simulink model "structure_track_side"  (R2026b)
settings: Solver=VariableStepAuto
model mask{side=1 left}
  mask prompts: side "Track side"
undefined symbols (not defined in the file or in its folder): P
libraries: fl_lib x11, nesl_utility x6
settings Model: Creator=aomar  LastModifiedBy=aomar

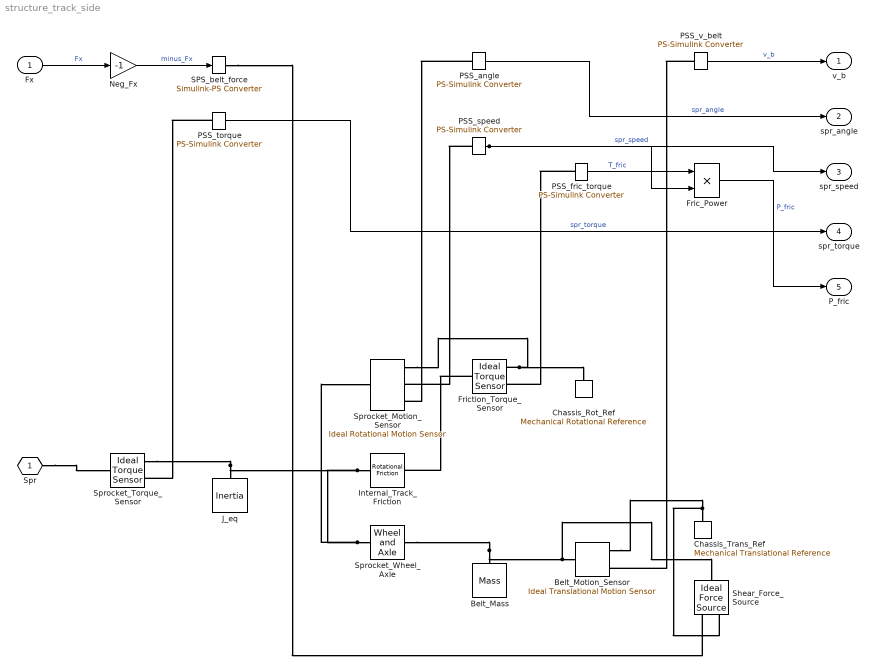
== system structure_track_side ==
  Fx : Inport
  Belt_Mass : fl_lib/Mechanical/Translational Elements/Mass  mass=P.structure.track.m_belt kg  num_ports=foundation.enum.numPorts2.one  v_specify=off  v_priority=High  v=0 m/s  v_nominal_specify=off  v_nominal_value=1  v_nominal_unit=m/s  f_specify=off  f_priority=None  f=0 N  f_nominal_specify=off  f_nominal_value=1  f_nominal_unit=N
  Belt_Motion_Sensor : fl_lib/Mechanical/Mechanical Sensors/Ideal Translational Motion Sensor  reference=foundation.enum.MeasurementReference.difference  acceleration_port=false  velocity_port=true  position_port=false  offset=0 m
  Chassis_Rot_Ref : fl_lib/Mechanical/Rotational Elements/Mechanical Rotational Reference
  Chassis_Trans_Ref : fl_lib/Mechanical/Translational Elements/Mechanical Translational Reference
  Fric_Power : Product  Inputs=**
  Friction_Torque_Sensor : fl_lib/Mechanical/Mechanical Sensors/Ideal Torque Sensor
  Internal_Track_Friction : fl_lib/Mechanical/Rotational Elements/Rotational Friction  brkwy_trq=P.structure.track.T_brk N*m  brkwy_vel=P.structure.track.w_brk rad/s  Col_trq=P.structure.track.T_col N*m  visc_coef=P.structure.track.c_visc N*m*s/rad  w_specify=off  w_priority=None  w=0 rad/s  w_nominal_specify=off  w_nominal_value=1  w_nominal_unit=rad/s  t_specify=off  t_priority=None  t=0 N*m  t_nominal_specify=off  t_nominal_value=1  t_nominal_unit=N*m
  J_eq : fl_lib/Mechanical/Rotational Elements/Inertia  inertia=P.structure.track.J_eq kg*m^2  num_ports=foundation.enum.numPorts2.one  w_specify=on  w_priority=High  w=P.structure.init.v0/P.structure.r_sprocket rad/s  w_nominal_specify=off  w_nominal_value=1  w_nominal_unit=rad/s  t_specify=off  t_priority=None  t=0 N*m  t_nominal_specify=off  t_nominal_value=1  t_nominal_unit=N*m
  Neg_Fx : Gain  Gain=-1
  PSS_angle : nesl_utility/PS-Simulink Converter  PhysicalDomain=network_engine_domain  SubClassName=ps_output  LeftPortType=input  RightPortType=output  PseudoPeriodic=off  Frequencies=[]  VectorFormat=inherit  Unit=rad  AffineConversion=off
  PSS_fric_torque : nesl_utility/PS-Simulink Converter  PhysicalDomain=network_engine_domain  SubClassName=ps_output  LeftPortType=input  RightPortType=output  PseudoPeriodic=off  Frequencies=[]  VectorFormat=inherit  Unit=N*m  AffineConversion=off
  PSS_speed : nesl_utility/PS-Simulink Converter  PhysicalDomain=network_engine_domain  SubClassName=ps_output  LeftPortType=input  RightPortType=output  PseudoPeriodic=off  Frequencies=[]  VectorFormat=inherit  Unit=rad/s  AffineConversion=off
  PSS_torque : nesl_utility/PS-Simulink Converter  PhysicalDomain=network_engine_domain  SubClassName=ps_output  LeftPortType=input  RightPortType=output  PseudoPeriodic=off  Frequencies=[]  VectorFormat=inherit  Unit=N*m  AffineConversion=off
  PSS_v_belt : nesl_utility/PS-Simulink Converter  PhysicalDomain=network_engine_domain  SubClassName=ps_output  LeftPortType=input  RightPortType=output  PseudoPeriodic=off  Frequencies=[]  VectorFormat=inherit  Unit=m/s  AffineConversion=off
  SPS_belt_force : nesl_utility/Simulink-PS Converter  PhysicalDomain=network_engine_domain  SubClassName=ps_input  LeftPortType=input  RightPortType=output  PseudoPeriodic=off  Frequencies=[]  NoiseDistribution=none  NoiseParameters=[]  Unit=N  AffineConversion=off  FilteringAndDerivatives=zero  SimscapeFilterOrder=1  InputFilterTimeConstant=0.001  UdotUserProvided=0
  Shear_Force_Source : fl_lib/Mechanical/Mechanical Sources/Ideal Force Source
  Sprocket_Motion_Sensor : fl_lib/Mechanical/Mechanical Sensors/Ideal Rotational Motion Sensor  reference=foundation.enum.MeasurementReference.difference  acceleration_port=false  velocity_port=true  position_port=true  wrap_angle=false  offset=0 rad
  Sprocket_Torque_Sensor : fl_lib/Mechanical/Mechanical Sensors/Ideal Torque Sensor
  Sprocket_Wheel_Axle : fl_lib/Mechanical/Mechanisms/Wheel and Axle  R=P.structure.r_sprocket m  or=foundation.enum.DriveOrientation.Positive  t_specify=off  t_priority=None  t=0 N*m  t_nominal_specify=off  t_nominal_value=1  t_nominal_unit=N*m  f_specify=off  f_priority=None  f=0 N  f_nominal_specify=off  f_nominal_value=1  f_nominal_unit=N
  Spr : PMIOPort  Side=Left  ConnectionType=Connection: foundation.mechanical.rotational.rotational
  v_b : Outport
  spr_angle : Outport  Port=2
  spr_speed : Outport  Port=3
  spr_torque : Outport  Port=4
  P_fric : Outport  Port=5
  wires:
  Fx/1 -> Neg_Fx/1  "Fx"
  Neg_Fx/1 -> SPS_belt_force/1  "minus_Fx"
  PSS_torque/1 -> spr_torque/1  "spr_torque"
  PSS_angle/1 -> spr_angle/1  "spr_angle"
  PSS_speed/1 -> Fric_Power/2, spr_speed/1  "spr_speed"
  PSS_fric_torque/1 -> Fric_Power/1  "T_fric"
  PSS_v_belt/1 -> v_b/1  "v_b"
  Fric_Power/1 -> P_fric/1  "P_fric"
  connections:
  Belt_Mass/LConn1 -- Sprocket_Wheel_Axle/RConn1 -- Belt_Motion_Sensor/LConn1 -- Shear_Force_Source/LConn1
  Chassis_Trans_Ref/LConn1 -- Belt_Motion_Sensor/RConn1 -- Shear_Force_Source/RConn2
  PSS_v_belt/LConn1 -- Belt_Motion_Sensor/RConn2
  Friction_Torque_Sensor/RConn1 -- Sprocket_Motion_Sensor/RConn1 -- Chassis_Rot_Ref/LConn1
  Friction_Torque_Sensor/LConn1 -- Internal_Track_Friction/RConn1
  PSS_fric_torque/LConn1 -- Friction_Torque_Sensor/RConn2
  J_eq/LConn1 -- Sprocket_Torque_Sensor/RConn1 -- Internal_Track_Friction/LConn1 -- Sprocket_Wheel_Axle/LConn1 -- Sprocket_Motion_Sensor/LConn1
  PSS_angle/LConn1 -- Sprocket_Motion_Sensor/RConn3
  PSS_speed/LConn1 -- Sprocket_Motion_Sensor/RConn2
  PSS_torque/LConn1 -- Sprocket_Torque_Sensor/RConn2
  SPS_belt_force/RConn1 -- Shear_Force_Source/RConn1
  Spr/RConn1 -- Sprocket_Torque_Sensor/LConn1
